simulink model "SZ05_ARM"  (R2026a)
settings: Solver=VariableStepAuto  MaxStep=tau/25
InitFcn:
  | K = 5;
  | tau = 0.125;
  | 
  | y_0 = 2.5;
libraries: MK_SZ x2
settings Model: Creator=Szalay  LastModifiedBy=Szalay

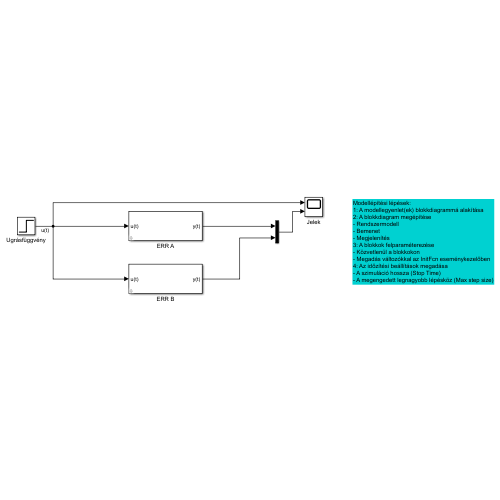
[thumbnail: Simulink's stored preview of the top-level diagram]
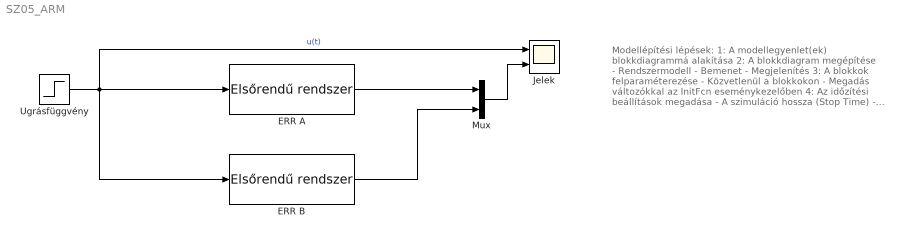
== system SZ05_ARM ==
  note: Modellépítési lépések:
      | 1: A modellegyenlet(ek) blokkdiagrammá alakítása
      | 2: A blokkdiagram megépítése
      | - Rendszermodell
      | - Bemenet
      | - Megjelenítés
      | 3: A blokkok felparaméterezése
      | - Közvetlenül a blokkokon
      | - Megadás változókkal az InitFcn eseménykezelőben
      | 4: Az időzítési beállítások megadása
      | - A szimuláció hossza (Stop Time)
      | - A megengedett legnagyobb lépésköz (Max step size)
  ERR A : MK_SZ/Elsőrendű rendszer  K=1  tau=1  y_0=0
  ERR B : MK_SZ/Elsőrendű rendszer  K=1  tau=1  y_0=0
  Jelek : Scope  NumInputPorts=2
      settings: ActiveDisplayYMinimum=-0.31249999999999994  ActiveDisplayYMaximum=2.8125
  Mux : Mux  Inputs=2
  Ugrásfüggvény : Step  Time=5  SampleTime=0
  wires:
  Ugrásfüggvény/1 -> ERR B/1, ERR A/1, Jelek/1  "u(t)"
  Mux/1 -> Jelek/2
  ERR A/1 -> Mux/1
  ERR B/1 -> Mux/2
